simulink model "Test2D_Disks_in_Box"  (R2024a)
settings: Solver=ode15s  StartTime=0.0  StopTime=3  MaxStep=1e-2  RelTol=1e-4  AbsTol=1e-5  EnableMultiTasking=on
PostLoadFcn:
  | warning off Simulink:Engine:UsingDefaultMaxStepSize
InitFcn:
  | k_contact = 1e4;
  | b_contact = 1e1;
StartFcn:
  | tic;
StopFcn:
  | Elapsed_Sim_Time = toc;
  | disp(['Elapsed Sim Time = ' num2str(Elapsed_Sim_Time)]);
model workspace (MATLAB code in the model file):
  | Disk.radius = 0.05;
  | Disk.length = 0.01;
  | Disk.density = 1000;
  | 
  | Box.outer_width = 0.51*2;
  | Box.inner_width = 0.49*2;
  | Box.width = 0.05;
undefined symbols (not defined in the file or in its folder): Extr_Data_Box, X, Y, Z
libraries: sm_lib x22, Contact_Forces_Lib x15, Parts_Lib x3, nesl_utility x2
CloseFcn:
  | try,close(h1_Test2D_Disks_in_Box),end
  | clear h1_Test2D_Disks_in_Box
  | 
  | clear simlog_Test2D_Disks_in_Box
  | clear logsout_Test2D_Disks_in_Box
Description:
  | Test Model Disks in Box
  | 
  | Copyright 2015-2024 The MathWorks, Inc.
settings Model: Creator=smiller  LastModifiedBy=smiller
settings SolverCC: AutoScaleAbsTol=off  AlgebraicLoopSolver=TrustRegion
settings DataIOCC: MaxDataPoints=10000  SaveFormat=Array  ReturnWorkspaceOutputs=off  SignalLoggingName=logsout_Test2D_Disks_in_Box
settings OptimizationCC: ReuseModelBlockBuffer=off  ExpressionDepthLimit=2147483647  LifeSpan=inf
settings DebuggingCC: AlgebraicLoopMsg=error  UnderspecifiedInitializationDetection=Classic  MergeDetectMultiDrivingBlocksExec=none  IgnoredZcDiagnostic=none  SolverPrmCheckMsg=warning  FcnCallInpInsideContextMsg=warning  UnconnectedInputMsg=warning  UnconnectedLineMsg=warning  AllowSymbolicDim=off  StateNameClashWarn=warning  PregeneratedLibrarySubsystemCodeDiagnostic=none  SFUnexpectedBacktrackingDiag=warning  SFNoUnconditionalDefaultTransitionDiag=warning  SFExecutionAtInitializationDiag=none  ArithmeticOperatorsInVariantConditions=warning
settings HardwareCC: ProdBitPerPointer=32  ProdBitPerSizeT=32  ProdBitPerPtrDiffT=32  ProdLargestAtomicFloat=None  ProdIntDivRoundTo=Undefined  ProdEndianess=Unspecified  ProdWordSize=32  ProdHWDeviceType=32-bit Generic
settings ModelReferenceCC: EnableRefExpFcnMdlSchedulingChecks=on  PropagateSignalLabelsOutOfModel=off
settings SFSimCC: SimUseLocalCustomCode=off  CustomCodeUndefinedFunction=UseInterfaceOnly
settings RTWCC: RTWUseLocalCustomCode=off  GPUComputeCapability=3.5  DLArmComputeVersion=19.05
settings CodeAppCC: StateflowObjectComments=on
settings GRTTargetCC: TargetLangStandard=C89/C90 (ANSI)
settings ConfigComp: CovMetricSettings=dw  CovSaveCumulativeToWorkspaceVar=on  CovSaveSingleToWorkspaceVar=on  CovExternalEMLEnable=off  CovSFcnEnable=off
settings SimscapeCC: SimscapeNormalizeSystem=off  SimscapeLogType=all  SimscapeLogSimulationStatistics=on  SimscapeLogName=simlog_Test2D_Disks_in_Box  SimscapeLogDataHistory=10000
settings ConfigurationSet: Description=SimMechanics 2G
settings DiagnosticsConfigSet: SimMechanicsRigidlyBoundBlock=none
settings ExplorerConfigSet: InternalSimMechanicsExplorerSettings="<ExplorerConfiguration><canonicalview>default</canonicalview><AnimationSetting><BasePlaybackSpeed>1.0</BasePlaybackSpeed><PlaybackSpeedFactor>1.0</PlaybackSpeedFactor></AnimationSetting><TilePanel><TileInfo><Tiles Columns=\"1\" Count=\"1\" Rows=\"1\"><Column Left=\"2\" Weight=\"1\"/><Column Left=\"635\"/><Row Top=\"2\" Weight=\"1\"/><Row Top=\"394\"/><Tile Height=\"1\" Width=\"1\" X=\"0\" Y=\"0\"/></Tiles></TileInfo><SceneInfo><SceneViewer><BGColor><R>0.90588235855102539</R><G>0.94117647409439087</G><B>0.94117647409439087</B></BGColor><Camera><DoPerspective>off</DoPerspective><Position><X>0</X><Y>-1.0218563054680825</Y><Z>2.2204460492503131e-16</Z></Position><Center><X>0</X><Y>-4.9303806576313238e-32</Y><Z>2.2204460492503131e-16</Z></Center><Up><X>0</X><Y>-0</Y><Z>1</Z></Up><ViewLimDist>1</ViewLimDist><YLim>0.52529999017715456</YLim><XLim>0.85584123725990713</XLim></Camera></SceneViewer></SceneInfo></TilePanel><MechEditorPanel><Cameras/><GfxPanelCameraMap/></MechEditorPanel></ExplorerConfiguration>"

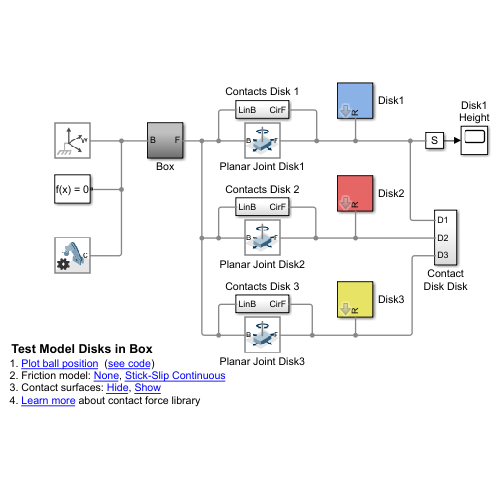
[thumbnail: Simulink's stored preview of the top-level diagram]
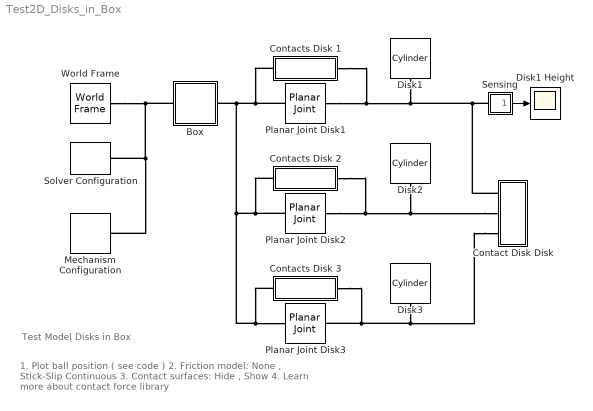
== system Test2D_Disks_in_Box ==
  note: 1. Plot ball position ( see code )
      | 2. Friction model: None , Stick-Slip Continuous
      | 3. Contact surfaces: Hide , Show
      | 4. Learn more about contact force library
  note: Test Model Disks in Box
  Box : Subsystem  Tag=CustomStyle
  Contact Disk Disk : Subsystem
  Contacts Disk 1 : Subsystem
  Contacts Disk 2 : Subsystem
  Contacts Disk 3 : Subsystem
  Disk1 : Parts_Lib/Cylinder  cyl_radius=Disk.radius  cyl_length=Disk.length  cyl_density=Disk.density  cyl_color=blue  cyl_opacity=1  cyl_color_custom="[0.7920    0.9900    0.9900]"  mark_radius=[0.75 0.5]  mark_len_factor=1.01  mark_angle=60  mark_color=orange  mark_opacity=1
  Disk1 Height : Scope
  Disk2 : Parts_Lib/Cylinder  cyl_radius=Disk.radius  cyl_length=Disk.length  cyl_density=Disk.density  cyl_color=red  cyl_opacity=1  cyl_color_custom="[0.7920    0.9900    0.9900]"  mark_radius=[0.75 0.5]  mark_len_factor=1.01  mark_angle=60  mark_color=green  mark_opacity=1
  Disk3 : Parts_Lib/Cylinder  cyl_radius=Disk.radius  cyl_length=Disk.length  cyl_density=Disk.density  cyl_color=yellow  cyl_opacity=1  cyl_color_custom="[0.7920    0.9900    0.9900]"  mark_radius=[0.75 0.5]  mark_len_factor=1.01  mark_angle=60  mark_color=purple  mark_opacity=1
  Mechanism Configuration : sm_lib/Utilities/Mechanism Configuration  UniformGravity=Constant  GravityVector=[0 0 -9.81]  GravityVectorUnits=m/s^2  LinearizationDelta=0.001  JointModeTransitionNonlinearIterations=2
  Planar Joint Disk1 : sm_lib/Joints/Planar Joint  JointMode=Normal  CompositeWrenchDir=FollowerOnBase  CompositeWrenchFrame=BaseFrame  SenseConstraintForce=off  SenseConstraintTorque=off  SenseTotalForce=off  SenseTotalTorque=off  PxPositionTargetSpecify=on  PxPositionTargetPriority=High  PxPositionTargetValue=0.3  PxPositionTargetValueUnits=m  PxVelocityTargetSpecify=on  PxVelocityTargetPriority=High  PxVelocityTargetValue=-1  PxVelocityTargetValueUnits=m/s  PxEquilibriumPosition=0  PxEquilibriumPositionUnits=m  PxSpringStiffness=0  PxSpringStiffnessUnits=N/m  PxDampingCoefficient=0  PxDampingCoefficientUnits=N/(m/s)  PxLowerLimitSpecify=off  PxLowerLimitBound=-1  PxLowerLimitBoundUnits=m  PxLowerLimitStiffness=1e6  PxLowerLimitStiffnessUnits=N/m  PxLowerLimitDamping=1e3  PxLowerLimitDampingUnits=N/(m/s)  PxLowerLimitTransitionRegionWidth=1e-4  PxLowerLimitTransitionRegionWidthUnits=m  PxUpperLimitSpecify=off  PxUpperLimitBound=1  PxUpperLimitBoundUnits=m  PxUpperLimitStiffness=1e6  PxUpperLimitStiffnessUnits=N/m  PxUpperLimitDamping=1e3  PxUpperLimitDampingUnits=N/(m/s)  PxUpperLimitTransitionRegionWidth=1e-4  PxUpperLimitTransitionRegionWidthUnits=m  PxTorqueActuationMode=NoTorque  PxMotionActuationMode=ComputedMotion  PxSensePosition=off  PxSenseVelocity=off  PxSenseAcceleration=off  PxSenseTorqueForce=off  PxSenseLowerLimitTorqueForce=off  PxSenseUpperLimitTorqueForce=off  PyPositionTargetSpecify=off  PyPositionTargetPriority=High  PyPositionTargetValue=0  PyPositionTargetValueUnits=m  PyVelocityTargetSpecify=on  PyVelocityTargetPriority=High  PyVelocityTargetValue=1  PyVelocityTargetValueUnits=m/s  PyEquilibriumPosition=0  PyEquilibriumPositionUnits=m  PySpringStiffness=0  PySpringStiffnessUnits=N/m  PyDampingCoefficient=0  PyDampingCoefficientUnits=N/(m/s)  PyLowerLimitSpecify=off  PyLowerLimitBound=-1  PyLowerLimitBoundUnits=m  PyLowerLimitStiffness=1e6  PyLowerLimitStiffnessUnits=N/m  PyLowerLimitDamping=1e3  PyLowerLimitDampingUnits=N/(m/s)  PyLowerLimitTransitionRegionWidth=1e-4  PyLowerLimitTransitionRegionWidthUnits=m  PyUpperLimitSpecify=off  PyUpperLimitBound=1  PyUpperLimitBoundUnits=m  PyUpperLimitStiffness=1e6  PyUpperLimitStiffnessUnits=N/m  PyUpperLimitDamping=1e3  PyUpperLimitDampingUnits=N/(m/s)  PyUpperLimitTransitionRegionWidth=1e-4  PyUpperLimitTransitionRegionWidthUnits=m  PyTorqueActuationMode=NoTorque  PyMotionActuationMode=ComputedMotion  PySensePosition=off  PySenseVelocity=off  PySenseAcceleration=off  PySenseTorqueForce=off  PySenseLowerLimitTorqueForce=off  PySenseUpperLimitTorqueForce=off  RzPositionTargetSpecify=off  RzPositionTargetPriority=High  RzPositionTargetValue=0  RzPositionTargetValueUnits=deg  RzVelocityTargetSpecify=off  RzVelocityTargetPriority=High  RzVelocityTargetValue=0  RzVelocityTargetValueUnits=deg/s  RzEquilibriumPosition=0  RzEquilibriumPositionUnits=deg  RzSpringStiffness=0  RzSpringStiffnessUnits=N*m/deg  RzDampingCoefficient=0  RzDampingCoefficientUnits=N*m/(deg/s)  RzLowerLimitSpecify=off  RzLowerLimitBound=-90  RzLowerLimitBoundUnits=deg  RzLowerLimitStiffness=1e4  RzLowerLimitStiffnessUnits=N*m/deg  RzLowerLimitDamping=10  RzLowerLimitDampingUnits=N*m/(deg/s)  RzLowerLimitTransitionRegionWidth=0.1  RzLowerLimitTransitionRegionWidthUnits=deg  RzUpperLimitSpecify=off  RzUpperLimitBound=90  RzUpperLimitBoundUnits=deg  RzUpperLimitStiffness=1e4  RzUpperLimitStiffnessUnits=N*m/deg  RzUpperLimitDamping=10  RzUpperLimitDampingUnits=N*m/(deg/s)  RzUpperLimitTransitionRegionWidth=0.1  RzUpperLimitTransitionRegionWidthUnits=deg  RzTorqueActuationMode=NoTorque  RzMotionActuationMode=ComputedMotion  RzSensePosition=off  RzSenseVelocity=off  RzSenseAcceleration=off  RzSenseTorqueForce=off  RzSenseLowerLimitTorqueForce=off  RzSenseUpperLimitTorqueForce=off
  Planar Joint Disk2 : sm_lib/Joints/Planar Joint  JointMode=Normal  CompositeWrenchDir=FollowerOnBase  CompositeWrenchFrame=BaseFrame  SenseConstraintForce=off  SenseConstraintTorque=off  SenseTotalForce=off  SenseTotalTorque=off  PxPositionTargetSpecify=on  PxPositionTargetPriority=High  PxPositionTargetValue=-0.3  PxPositionTargetValueUnits=m  PxVelocityTargetSpecify=on  PxVelocityTargetPriority=High  PxVelocityTargetValue=+1  PxVelocityTargetValueUnits=m/s  PxEquilibriumPosition=0  PxEquilibriumPositionUnits=m  PxSpringStiffness=0  PxSpringStiffnessUnits=N/m  PxDampingCoefficient=0  PxDampingCoefficientUnits=N/(m/s)  PxLowerLimitSpecify=off  PxLowerLimitBound=-1  PxLowerLimitBoundUnits=m  PxLowerLimitStiffness=1e6  PxLowerLimitStiffnessUnits=N/m  PxLowerLimitDamping=1e3  PxLowerLimitDampingUnits=N/(m/s)  PxLowerLimitTransitionRegionWidth=1e-4  PxLowerLimitTransitionRegionWidthUnits=m  PxUpperLimitSpecify=off  PxUpperLimitBound=1  PxUpperLimitBoundUnits=m  PxUpperLimitStiffness=1e6  PxUpperLimitStiffnessUnits=N/m  PxUpperLimitDamping=1e3  PxUpperLimitDampingUnits=N/(m/s)  PxUpperLimitTransitionRegionWidth=1e-4  PxUpperLimitTransitionRegionWidthUnits=m  PxTorqueActuationMode=NoTorque  PxMotionActuationMode=ComputedMotion  PxSensePosition=off  PxSenseVelocity=off  PxSenseAcceleration=off  PxSenseTorqueForce=off  PxSenseLowerLimitTorqueForce=off  PxSenseUpperLimitTorqueForce=off  PyPositionTargetSpecify=off  PyPositionTargetPriority=High  PyPositionTargetValue=0  PyPositionTargetValueUnits=m  PyVelocityTargetSpecify=on  PyVelocityTargetPriority=High  PyVelocityTargetValue=-0.8  PyVelocityTargetValueUnits=m/s  PyEquilibriumPosition=0  PyEquilibriumPositionUnits=m  PySpringStiffness=0  PySpringStiffnessUnits=N/m  PyDampingCoefficient=0  PyDampingCoefficientUnits=N/(m/s)  PyLowerLimitSpecify=off  PyLowerLimitBound=-1  PyLowerLimitBoundUnits=m  PyLowerLimitStiffness=1e6  PyLowerLimitStiffnessUnits=N/m  PyLowerLimitDamping=1e3  PyLowerLimitDampingUnits=N/(m/s)  PyLowerLimitTransitionRegionWidth=1e-4  PyLowerLimitTransitionRegionWidthUnits=m  PyUpperLimitSpecify=off  PyUpperLimitBound=1  PyUpperLimitBoundUnits=m  PyUpperLimitStiffness=1e6  PyUpperLimitStiffnessUnits=N/m  PyUpperLimitDamping=1e3  PyUpperLimitDampingUnits=N/(m/s)  PyUpperLimitTransitionRegionWidth=1e-4  PyUpperLimitTransitionRegionWidthUnits=m  PyTorqueActuationMode=NoTorque  PyMotionActuationMode=ComputedMotion  PySensePosition=off  PySenseVelocity=off  PySenseAcceleration=off  PySenseTorqueForce=off  PySenseLowerLimitTorqueForce=off  PySenseUpperLimitTorqueForce=off  RzPositionTargetSpecify=off  RzPositionTargetPriority=High  RzPositionTargetValue=0  RzPositionTargetValueUnits=deg  RzVelocityTargetSpecify=off  RzVelocityTargetPriority=High  RzVelocityTargetValue=0  RzVelocityTargetValueUnits=deg/s  RzEquilibriumPosition=0  RzEquilibriumPositionUnits=deg  RzSpringStiffness=0  RzSpringStiffnessUnits=N*m/deg  RzDampingCoefficient=0  RzDampingCoefficientUnits=N*m/(deg/s)  RzLowerLimitSpecify=off  RzLowerLimitBound=-90  RzLowerLimitBoundUnits=deg  RzLowerLimitStiffness=1e4  RzLowerLimitStiffnessUnits=N*m/deg  RzLowerLimitDamping=10  RzLowerLimitDampingUnits=N*m/(deg/s)  RzLowerLimitTransitionRegionWidth=0.1  RzLowerLimitTransitionRegionWidthUnits=deg  RzUpperLimitSpecify=off  RzUpperLimitBound=90  RzUpperLimitBoundUnits=deg  RzUpperLimitStiffness=1e4  RzUpperLimitStiffnessUnits=N*m/deg  RzUpperLimitDamping=10  RzUpperLimitDampingUnits=N*m/(deg/s)  RzUpperLimitTransitionRegionWidth=0.1  RzUpperLimitTransitionRegionWidthUnits=deg  RzTorqueActuationMode=NoTorque  RzMotionActuationMode=ComputedMotion  RzSensePosition=off  RzSenseVelocity=off  RzSenseAcceleration=off  RzSenseTorqueForce=off  RzSenseLowerLimitTorqueForce=off  RzSenseUpperLimitTorqueForce=off
  Planar Joint Disk3 : sm_lib/Joints/Planar Joint  JointMode=Normal  CompositeWrenchDir=FollowerOnBase  CompositeWrenchFrame=BaseFrame  SenseConstraintForce=off  SenseConstraintTorque=off  SenseTotalForce=off  SenseTotalTorque=off  PxPositionTargetSpecify=off  PxPositionTargetPriority=High  PxPositionTargetValue=0  PxPositionTargetValueUnits=m  PxVelocityTargetSpecify=on  PxVelocityTargetPriority=High  PxVelocityTargetValue=+1  PxVelocityTargetValueUnits=m/s  PxEquilibriumPosition=0  PxEquilibriumPositionUnits=m  PxSpringStiffness=0  PxSpringStiffnessUnits=N/m  PxDampingCoefficient=0  PxDampingCoefficientUnits=N/(m/s)  PxLowerLimitSpecify=off  PxLowerLimitBound=-1  PxLowerLimitBoundUnits=m  PxLowerLimitStiffness=1e6  PxLowerLimitStiffnessUnits=N/m  PxLowerLimitDamping=1e3  PxLowerLimitDampingUnits=N/(m/s)  PxLowerLimitTransitionRegionWidth=1e-4  PxLowerLimitTransitionRegionWidthUnits=m  PxUpperLimitSpecify=off  PxUpperLimitBound=1  PxUpperLimitBoundUnits=m  PxUpperLimitStiffness=1e6  PxUpperLimitStiffnessUnits=N/m  PxUpperLimitDamping=1e3  PxUpperLimitDampingUnits=N/(m/s)  PxUpperLimitTransitionRegionWidth=1e-4  PxUpperLimitTransitionRegionWidthUnits=m  PxTorqueActuationMode=NoTorque  PxMotionActuationMode=ComputedMotion  PxSensePosition=off  PxSenseVelocity=off  PxSenseAcceleration=off  PxSenseTorqueForce=off  PxSenseLowerLimitTorqueForce=off  PxSenseUpperLimitTorqueForce=off  PyPositionTargetSpecify=on  PyPositionTargetPriority=High  PyPositionTargetValue=0.3  PyPositionTargetValueUnits=m  PyVelocityTargetSpecify=on  PyVelocityTargetPriority=High  PyVelocityTargetValue=-0.8  PyVelocityTargetValueUnits=m/s  PyEquilibriumPosition=0  PyEquilibriumPositionUnits=m  PySpringStiffness=0  PySpringStiffnessUnits=N/m  PyDampingCoefficient=0  PyDampingCoefficientUnits=N/(m/s)  PyLowerLimitSpecify=off  PyLowerLimitBound=-1  PyLowerLimitBoundUnits=m  PyLowerLimitStiffness=1e6  PyLowerLimitStiffnessUnits=N/m  PyLowerLimitDamping=1e3  PyLowerLimitDampingUnits=N/(m/s)  PyLowerLimitTransitionRegionWidth=1e-4  PyLowerLimitTransitionRegionWidthUnits=m  PyUpperLimitSpecify=off  PyUpperLimitBound=1  PyUpperLimitBoundUnits=m  PyUpperLimitStiffness=1e6  PyUpperLimitStiffnessUnits=N/m  PyUpperLimitDamping=1e3  PyUpperLimitDampingUnits=N/(m/s)  PyUpperLimitTransitionRegionWidth=1e-4  PyUpperLimitTransitionRegionWidthUnits=m  PyTorqueActuationMode=NoTorque  PyMotionActuationMode=ComputedMotion  PySensePosition=off  PySenseVelocity=off  PySenseAcceleration=off  PySenseTorqueForce=off  PySenseLowerLimitTorqueForce=off  PySenseUpperLimitTorqueForce=off  RzPositionTargetSpecify=off  RzPositionTargetPriority=High  RzPositionTargetValue=0  RzPositionTargetValueUnits=deg  RzVelocityTargetSpecify=off  RzVelocityTargetPriority=High  RzVelocityTargetValue=0  RzVelocityTargetValueUnits=deg/s  RzEquilibriumPosition=0  RzEquilibriumPositionUnits=deg  RzSpringStiffness=0  RzSpringStiffnessUnits=N*m/deg  RzDampingCoefficient=0  RzDampingCoefficientUnits=N*m/(deg/s)  RzLowerLimitSpecify=off  RzLowerLimitBound=-90  RzLowerLimitBoundUnits=deg  RzLowerLimitStiffness=1e4  RzLowerLimitStiffnessUnits=N*m/deg  RzLowerLimitDamping=10  RzLowerLimitDampingUnits=N*m/(deg/s)  RzLowerLimitTransitionRegionWidth=0.1  RzLowerLimitTransitionRegionWidthUnits=deg  RzUpperLimitSpecify=off  RzUpperLimitBound=90  RzUpperLimitBoundUnits=deg  RzUpperLimitStiffness=1e4  RzUpperLimitStiffnessUnits=N*m/deg  RzUpperLimitDamping=10  RzUpperLimitDampingUnits=N*m/(deg/s)  RzUpperLimitTransitionRegionWidth=0.1  RzUpperLimitTransitionRegionWidthUnits=deg  RzTorqueActuationMode=NoTorque  RzMotionActuationMode=ComputedMotion  RzSensePosition=off  RzSenseVelocity=off  RzSenseAcceleration=off  RzSenseTorqueForce=off  RzSenseLowerLimitTorqueForce=off  RzSenseUpperLimitTorqueForce=off
  Sensing : Subsystem
      mask Display: disp('S')
  Solver Configuration : nesl_utility/Solver Configuration  PhysicalDomain=network_engine_domain  SubClassName=solver  LeftPortType=input  RightPortType=generic  Tones=[]  Harmonics=[]  SimulateNoise=off  Profile=off  UseLocalSampling=off  EnableSwitchedLinearOptims=on  FrequencyDomain=off  UseCCode=off  RelTol=0.001  AbsTol=1e-06  MinStep=1e-09  ToWorkspace=off  RevertToSquareIcSolve=off  NumHomotopyIterations=100  PhasorMode=off  PhasorModeNumHarmonics=1  ConsistencySolver=NEWTON_FTOL  IndexReductionMethod=DerivativeReplacement  DoDC=off  ResidualTolerance=1e-9  ConsistencyTolSource=GLOBAL  ConsistencyAbsTol=0.001  ConsistencyRelTol=0.001  ConsistencyTolFactor=0.001  UseLocalSolver=off  LocalSolverChoice=NE_BACKWARD_EULER_ADVANCER  ResolveIndetEquations=on  FunctionEvalNumThread=1  LocalSolverSampleTime=.001  DoFixedCost=off  MaxNonlinIter=3  MaxModeIter=2  ComputeImpulses=off  ImpulseIterations=2  LinearAlgebra=Sparse  LinearAlgebraNumThread=0  EquationFormulation=NE_TIME_EF  DelaysMemoryBudget=1024  AutomaticFiltering=on  FilteringTimeConstant=0.001  PartitionStorageMethod=AS_NEEDED  PartitionMemoryBudget=1024  PartitionMethod=FAST  MultibodyUseLocalSolver=off  MultibodyLocalSolverChoice=ODE1  MultibodyLocalSolverSampleTime=0.001
  World Frame : sm_lib/Frames and Transforms/World Frame
  wires:
  Sensing/1(S) -> Disk1 Height/1
  connections:
  Contact Disk Disk/LConn2 -- Disk2/LConn1 -- Contacts Disk 2/LConn1 -- Planar Joint Disk2/RConn1
  Contact Disk Disk/LConn1 -- Disk1/LConn1 -- Contacts Disk 1/LConn1 -- Planar Joint Disk1/RConn1 -- Sensing/LConn1
  Mechanism Configuration/RConn1 -- Solver Configuration/RConn1 -- Box/LConn1 -- World Frame/RConn1
  Contact Disk Disk/LConn3 -- Disk3/LConn1 -- Contacts Disk 3/LConn1 -- Planar Joint Disk3/RConn1
  Planar Joint Disk1/LConn1 -- Contacts Disk 1/RConn1 -- Contacts Disk 3/RConn1 -- Planar Joint Disk3/LConn1 -- Contacts Disk 2/RConn1 -- Planar Joint Disk2/LConn1 -- Box/RConn1

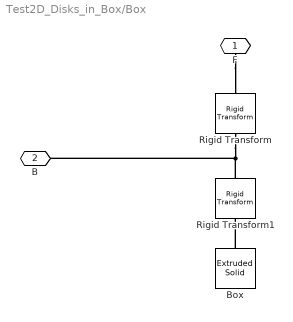
== system Test2D_Disks_in_Box/Box ==
  Box : sm_lib/Body Elements/Extruded Solid  ExtrusionType=General  PolygonNumSides=3  PolygonOuterRadius=1  PolygonOuterRadiusUnits=m  ExportEntireGeometry=off  ExtrusionCrossSection=Extr_Data_Box(Box.outer_width,Box.inner_width)  ExtrusionCrossSectionUnits=m  ExportConvexHullGeometry=off  ExtrusionLength=Box.width  ExtrusionLengthUnits=m  InertiaType=CalculateFromGeometry  BasedOnType=Density  Density=1000  DensityUnits=kg/(m^3)  Mass=1  MassUnits=kg  CenterOfMass=[0 0 0]  CenterOfMassUnits=m  MomentsOfInertia=[1 1 1]  MomentsOfInertiaUnits=kg*m^2  ProductsOfInertia=[0 0 0]  ProductsOfInertiaUnits=kg*m^2  GraphicType=FromGeometry  MarkerShape=Sphere  MarkerSize=10  GraphicVisPropType=SimpleVisualProperties  GraphicDiffuseColor=[0.5 0.5 0.5]  GraphicOpacity=1.0  GraphicSpecularColor=[0.5 0.5 0.5 1.0]  GraphicAmbientColor=[0.15 0.15 0.15 1.0]  GraphicEmissiveColor=[0.0 0.0 0.0 1.0]  GraphicShininess=75  DoExposeReferenceFrame=on  SerializedFrames=<Frames/>
  Rigid Transform : sm_lib/Frames and Transforms/Rigid Transform  RotationMethod=AlignedAxes  FollAlignAxisA=+X  BaseAlignAxisA=+Z  FollAlignAxisB=+Y  BaseAlignAxisB=+X  RotationStandardAxis=+Z  RotationAngle=0  RotationAngleUnits=deg  RotationArbitraryAxis=[0 0 1]  RotationSequenceAxes=FollowerAxes  RotationSequence=XYX  RotationSequenceAngles=[0 0 0]  RotationSequenceAnglesUnits=deg  RotationMatrix=[1 0 0; 0 1 0; 0 0 1]  Quaternion=[1 0 0 0]  TranslationMethod=None  TranslationCartesianOffset=[0 0 0]  TranslationCartesianOffsetUnits=m  TranslationStandardAxis=+Z  TranslationStandardOffset=0  TranslationStandardOffsetUnits=m  TranslationROffset=0  TranslationROffsetUnits=m  TranslationThetaOffset=0  TranslationThetaOffsetUnits=deg  TranslationZOffset=0  TranslationZOffsetUnits=m
  Rigid Transform1 : sm_lib/Frames and Transforms/Rigid Transform  RotationMethod=StandardAxis  FollAlignAxisA=+X  BaseAlignAxisA=+Z  FollAlignAxisB=+Y  BaseAlignAxisB=+X  RotationStandardAxis=+X  RotationAngle=90  RotationAngleUnits=deg  RotationArbitraryAxis=[0 0 1]  RotationSequenceAxes=FollowerAxes  RotationSequence=XYX  RotationSequenceAngles=[0 0 0]  RotationSequenceAnglesUnits=deg  RotationMatrix=[1 0 0; 0 1 0; 0 0 1]  Quaternion=[1 0 0 0]  TranslationMethod=None  TranslationCartesianOffset=[0 0 0]  TranslationCartesianOffsetUnits=m  TranslationStandardAxis=+Z  TranslationStandardOffset=0  TranslationStandardOffsetUnits=m  TranslationROffset=0  TranslationROffsetUnits=m  TranslationThetaOffset=0  TranslationThetaOffsetUnits=deg  TranslationZOffset=0  TranslationZOffsetUnits=m
  F : PMIOPort  Side=Right
  B : PMIOPort  Port=2  Side=Left
  connections:
  F/RConn1 -- Rigid Transform/RConn1
  Box/RConn1 -- Rigid Transform1/RConn1
  Rigid Transform/LConn1 -- B/RConn1 -- Rigid Transform1/LConn1

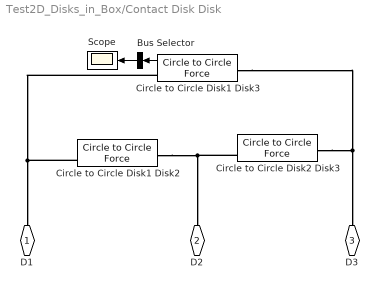
== system Test2D_Disks_in_Box/Contact Disk Disk ==
  Bus Selector : BusSelector  OutputSignals=Spr Force,Damp Force  OutputAsBus=on
  Circle to Circle Disk1 Disk2 : Contact_Forces_Lib/2D/Circle to Circle Force  cirB_rad=Disk.radius  cirF_rad=Disk.radius  active_angle=[-180 180]  force_law=Linear  k_contact=k_contact  b_contact=b_contact  pen_full_damp_F=1e-4  pen_exponent=1  custom_param_1=1  custom_param_2=1  friction_law=None  mu_kinetic=0.5  mu_static=0.7  v_thr=0.001  vis_on=off  vis_opc_en=0  vis_len_cirBz=Disk.length*1.05  vis_len_cirBx=Disk.radius*0.05  vis_len_cirFz=Disk.length*1.05  vis_len_cirFx=Disk.radius*0.05  vis_clr=[0.9 0.2 0.2]  vis_opc=0.7
  Circle to Circle Disk1 Disk3 : Contact_Forces_Lib/2D/Circle to Circle Force  cirB_rad=Disk.radius  cirF_rad=Disk.radius  active_angle=[-180 180]  force_law=Linear  k_contact=k_contact  b_contact=b_contact  pen_full_damp_F=1e-4  pen_exponent=1  custom_param_1=1  custom_param_2=1  friction_law=None  mu_kinetic=0.5  mu_static=0.7  v_thr=0.001  vis_on=off  vis_opc_en=0  vis_len_cirBz=Disk.length*1.05  vis_len_cirBx=Disk.radius*0.05  vis_len_cirFz=Disk.length*1.05  vis_len_cirFx=Disk.radius*0.05  vis_clr=[0.9 0.2 0.2]  vis_opc=0.7
  Circle to Circle Disk2 Disk3 : Contact_Forces_Lib/2D/Circle to Circle Force  cirB_rad=Disk.radius  cirF_rad=Disk.radius  active_angle=[-180 180]  force_law=Linear  k_contact=k_contact  b_contact=b_contact  pen_full_damp_F=1e-4  pen_exponent=1  custom_param_1=1  custom_param_2=1  friction_law=None  mu_kinetic=0.5  mu_static=0.7  v_thr=0.001  vis_on=off  vis_opc_en=0  vis_len_cirBz=Disk.length*1.05  vis_len_cirBx=Disk.radius*0.05  vis_len_cirFz=Disk.length*1.05  vis_len_cirFx=Disk.radius*0.05  vis_clr=[0.9 0.2 0.2]  vis_opc=0.7
  Scope : Scope
  D1 : PMIOPort  Side=Left
  D2 : PMIOPort  Port=2  Side=Left
  D3 : PMIOPort  Port=3  Side=Left
  wires:
  Circle to Circle Disk1 Disk3/1 -> Bus Selector/1
  Bus Selector/1 -> Scope/1
  connections:
  Circle to Circle Disk1 Disk3/RConn1 -- Circle to Circle Disk1 Disk2/RConn1 -- D1/RConn1
  Circle to Circle Disk2 Disk3/RConn1 -- Circle to Circle Disk1 Disk2/LConn1 -- D2/RConn1
  Circle to Circle Disk2 Disk3/LConn1 -- Circle to Circle Disk1 Disk3/LConn1 -- D3/RConn1

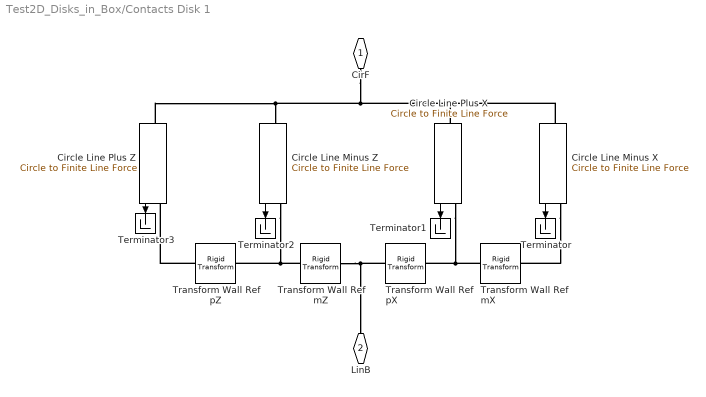
== system Test2D_Disks_in_Box/Contacts Disk 1 ==
  Circle Line Minus X : Contact_Forces_Lib/2D/Circle to Finite Line Force  circle_rad=Disk.radius  line_depth=(Box.outer_width/2-Box.inner_width/2)/2  line_length=(Box.outer_width+Box.inner_width)/2  force_law=Linear  k_contact=k_contact  b_contact=b_contact  pen_full_damp_F=1e-4  pen_exponent=1  custom_param_1=1  custom_param_2=1  friction_law=None  mu_kinetic=0.5  mu_static=0.7  v_thr=0.001  vis_on=off  vis_opc_en=0  vis_len_linBz=Box.width*1.05  vis_len_linBx=Box.outer_width*0.005  vis_len_cirFz=Disk.length*1.05  vis_len_cirFx=Disk.radius*0.05  vis_clr=[0.9 0.2 0.2]  vis_opc=0.7
  Circle Line Minus Z : Contact_Forces_Lib/2D/Circle to Finite Line Force  circle_rad=Disk.radius  line_depth=(Box.outer_width/2-Box.inner_width/2)/2  line_length=(Box.outer_width+Box.inner_width)/2  force_law=Linear  k_contact=k_contact  b_contact=b_contact  pen_full_damp_F=1e-4  pen_exponent=1  custom_param_1=1  custom_param_2=1  friction_law=None  mu_kinetic=0.5  mu_static=0.7  v_thr=0.001  vis_on=off  vis_opc_en=0  vis_len_linBz=Box.width*1.05  vis_len_linBx=Box.outer_width*0.005  vis_len_cirFz=Disk.length*1.05  vis_len_cirFx=Disk.radius*0.05  vis_clr=[0.9 0.2 0.2]  vis_opc=0.7
  Circle Line Plus X : Contact_Forces_Lib/2D/Circle to Finite Line Force  circle_rad=Disk.radius  line_depth=(Box.outer_width/2-Box.inner_width/2)/2  line_length=(Box.outer_width+Box.inner_width)/2  force_law=Linear  k_contact=k_contact  b_contact=b_contact  pen_full_damp_F=1e-4  pen_exponent=1  custom_param_1=1  custom_param_2=1  friction_law=None  mu_kinetic=0.5  mu_static=0.7  v_thr=0.001  vis_on=off  vis_opc_en=0  vis_len_linBz=Box.width*1.05  vis_len_linBx=Box.outer_width*0.005  vis_len_cirFz=Disk.length*1.05  vis_len_cirFx=Disk.radius*0.05  vis_clr=[0.9 0.2 0.2]  vis_opc=0.7
  Circle Line Plus Z : Contact_Forces_Lib/2D/Circle to Finite Line Force  circle_rad=Disk.radius  line_depth=(Box.outer_width/2-Box.inner_width/2)/2  line_length=(Box.outer_width+Box.inner_width)/2  force_law=Linear  k_contact=k_contact  b_contact=b_contact  pen_full_damp_F=1e-4  pen_exponent=1  custom_param_1=1  custom_param_2=1  friction_law=None  mu_kinetic=0.5  mu_static=0.7  v_thr=0.001  vis_on=off  vis_opc_en=0  vis_len_linBz=Box.width*1.05  vis_len_linBx=Box.outer_width*0.005  vis_len_cirFz=Disk.length*1.05  vis_len_cirFx=Disk.radius*0.05  vis_clr=[0.9 0.2 0.2]  vis_opc=0.7
  Terminator{,1..3} (4 alike) : Terminator
  Transform Wall Ref mX : sm_lib/Frames and Transforms/Rigid Transform  RotationMethod=StandardAxis  FollAlignAxisA=+X  BaseAlignAxisA=+Y  FollAlignAxisB=+Y  BaseAlignAxisB=+Z  RotationStandardAxis=+Z  RotationAngle=180  RotationAngleUnits=deg  RotationArbitraryAxis=[0 0 1]  RotationSequenceAxes=FollowerAxes  RotationSequence=XYX  RotationSequenceAngles=[0 0 0]  RotationSequenceAnglesUnits=deg  RotationMatrix=[1 0 0; 0 1 0; 0 0 1]  Quaternion=[1 0 0 0]  TranslationMethod=StandardAxis  TranslationCartesianOffset=[0 0 0]  TranslationCartesianOffsetUnits=m  TranslationStandardAxis=+X  TranslationStandardOffset=1  TranslationStandardOffsetUnits=m  TranslationROffset=0  TranslationROffsetUnits=m  TranslationThetaOffset=0  TranslationThetaOffsetUnits=deg  TranslationZOffset=0  TranslationZOffsetUnits=m
  Transform Wall Ref mZ : sm_lib/Frames and Transforms/Rigid Transform  RotationMethod=None  FollAlignAxisA=+X  BaseAlignAxisA=+Y  FollAlignAxisB=+Y  BaseAlignAxisB=+Z  RotationStandardAxis=+Z  RotationAngle=180  RotationAngleUnits=deg  RotationArbitraryAxis=[0 0 1]  RotationSequenceAxes=FollowerAxes  RotationSequence=XYX  RotationSequenceAngles=[0 0 0]  RotationSequenceAnglesUnits=deg  RotationMatrix=[1 0 0; 0 1 0; 0 0 1]  Quaternion=[1 0 0 0]  TranslationMethod=StandardAxis  TranslationCartesianOffset=[0 0 0]  TranslationCartesianOffsetUnits=m  TranslationStandardAxis=+X  TranslationStandardOffset=-0.5  TranslationStandardOffsetUnits=m  TranslationROffset=0  TranslationROffsetUnits=m  TranslationThetaOffset=0  TranslationThetaOffsetUnits=deg  TranslationZOffset=0  TranslationZOffsetUnits=m
  Transform Wall Ref pX : sm_lib/Frames and Transforms/Rigid Transform  RotationMethod=StandardAxis  FollAlignAxisA=+X  BaseAlignAxisA=+Y  FollAlignAxisB=+Y  BaseAlignAxisB=+Z  RotationStandardAxis=+Z  RotationAngle=-90  RotationAngleUnits=deg  RotationArbitraryAxis=[0 0 1]  RotationSequenceAxes=FollowerAxes  RotationSequence=XYX  RotationSequenceAngles=[0 0 0]  RotationSequenceAnglesUnits=deg  RotationMatrix=[1 0 0; 0 1 0; 0 0 1]  Quaternion=[1 0 0 0]  TranslationMethod=StandardAxis  TranslationCartesianOffset=[0 0 0]  TranslationCartesianOffsetUnits=m  TranslationStandardAxis=+Y  TranslationStandardOffset=0.5  TranslationStandardOffsetUnits=m  TranslationROffset=0  TranslationROffsetUnits=m  TranslationThetaOffset=0  TranslationThetaOffsetUnits=deg  TranslationZOffset=0  TranslationZOffsetUnits=m
  Transform Wall Ref pZ : sm_lib/Frames and Transforms/Rigid Transform  RotationMethod=StandardAxis  FollAlignAxisA=+X  BaseAlignAxisA=+Y  FollAlignAxisB=+Y  BaseAlignAxisB=+Z  RotationStandardAxis=+Z  RotationAngle=180  RotationAngleUnits=deg  RotationArbitraryAxis=[0 0 1]  RotationSequenceAxes=FollowerAxes  RotationSequence=XYX  RotationSequenceAngles=[0 0 0]  RotationSequenceAnglesUnits=deg  RotationMatrix=[1 0 0; 0 1 0; 0 0 1]  Quaternion=[1 0 0 0]  TranslationMethod=StandardAxis  TranslationCartesianOffset=[0 0 0]  TranslationCartesianOffsetUnits=m  TranslationStandardAxis=+X  TranslationStandardOffset=1  TranslationStandardOffsetUnits=m  TranslationROffset=0  TranslationROffsetUnits=m  TranslationThetaOffset=0  TranslationThetaOffsetUnits=deg  TranslationZOffset=0  TranslationZOffsetUnits=m
  CirF : PMIOPort  Side=Left
  LinB : PMIOPort  Port=2  Side=Right
  wires:
  Circle Line Minus Z/1 -> Terminator2/1
  Circle Line Minus X/1 -> Terminator/1
  Circle Line Plus X/1 -> Terminator1/1
  Circle Line Plus Z/1 -> Terminator3/1
  connections:
  CirF/RConn1 -- Circle Line Minus X/LConn1 -- Circle Line Plus X/LConn1 -- Circle Line Plus Z/LConn1 -- Circle Line Minus Z/LConn1
  Circle Line Minus Z/RConn1 -- Transform Wall Ref pZ/LConn1 -- Transform Wall Ref mZ/RConn1
  Transform Wall Ref pZ/RConn1 -- Circle Line Plus Z/RConn1
  Transform Wall Ref mZ/LConn1 -- Transform Wall Ref pX/LConn1 -- LinB/RConn1
  Circle Line Plus X/RConn1 -- Transform Wall Ref mX/LConn1 -- Transform Wall Ref pX/RConn1
  Circle Line Minus X/RConn1 -- Transform Wall Ref mX/RConn1

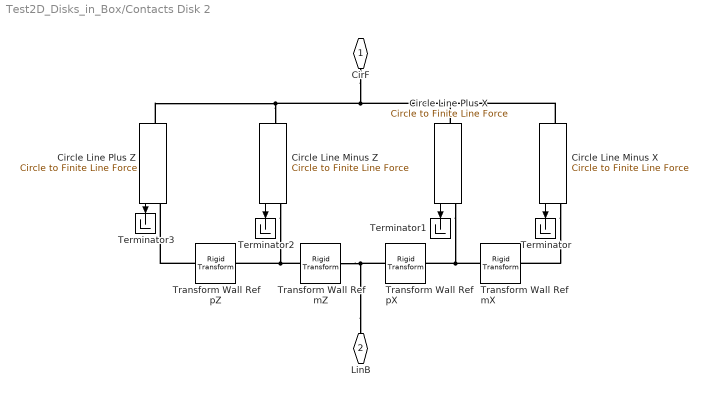
== system Test2D_Disks_in_Box/Contacts Disk 2 ==
  Circle Line Minus X : Contact_Forces_Lib/2D/Circle to Finite Line Force  circle_rad=Disk.radius  line_depth=(Box.outer_width/2-Box.inner_width/2)/2  line_length=(Box.outer_width+Box.inner_width)/2  force_law=Linear  k_contact=k_contact  b_contact=b_contact  pen_full_damp_F=1e-4  pen_exponent=1  custom_param_1=1  custom_param_2=1  friction_law=None  mu_kinetic=0.5  mu_static=0.7  v_thr=0.001  vis_on=off  vis_opc_en=0  vis_len_linBz=Box.width*1.05  vis_len_linBx=Box.outer_width*0.005  vis_len_cirFz=Disk.length*1.05  vis_len_cirFx=Disk.radius*0.05  vis_clr=[0.9 0.2 0.2]  vis_opc=0.7
  Circle Line Minus Z : Contact_Forces_Lib/2D/Circle to Finite Line Force  circle_rad=Disk.radius  line_depth=(Box.outer_width/2-Box.inner_width/2)/2  line_length=(Box.outer_width+Box.inner_width)/2  force_law=Linear  k_contact=k_contact  b_contact=b_contact  pen_full_damp_F=1e-4  pen_exponent=1  custom_param_1=1  custom_param_2=1  friction_law=None  mu_kinetic=0.5  mu_static=0.7  v_thr=0.001  vis_on=off  vis_opc_en=0  vis_len_linBz=Box.width*1.05  vis_len_linBx=Box.outer_width*0.005  vis_len_cirFz=Disk.length*1.05  vis_len_cirFx=Disk.radius*0.05  vis_clr=[0.9 0.2 0.2]  vis_opc=0.7
  Circle Line Plus X : Contact_Forces_Lib/2D/Circle to Finite Line Force  circle_rad=Disk.radius  line_depth=(Box.outer_width/2-Box.inner_width/2)/2  line_length=(Box.outer_width+Box.inner_width)/2  force_law=Linear  k_contact=k_contact  b_contact=b_contact  pen_full_damp_F=1e-4  pen_exponent=1  custom_param_1=1  custom_param_2=1  friction_law=None  mu_kinetic=0.5  mu_static=0.7  v_thr=0.001  vis_on=off  vis_opc_en=0  vis_len_linBz=Box.width*1.05  vis_len_linBx=Box.outer_width*0.005  vis_len_cirFz=Disk.length*1.05  vis_len_cirFx=Disk.radius*0.05  vis_clr=[0.9 0.2 0.2]  vis_opc=0.7
  Circle Line Plus Z : Contact_Forces_Lib/2D/Circle to Finite Line Force  circle_rad=Disk.radius  line_depth=(Box.outer_width/2-Box.inner_width/2)/2  line_length=(Box.outer_width+Box.inner_width)/2  force_law=Linear  k_contact=k_contact  b_contact=b_contact  pen_full_damp_F=1e-4  pen_exponent=1  custom_param_1=1  custom_param_2=1  friction_law=None  mu_kinetic=0.5  mu_static=0.7  v_thr=0.001  vis_on=off  vis_opc_en=0  vis_len_linBz=Box.width*1.05  vis_len_linBx=Box.outer_width*0.005  vis_len_cirFz=Disk.length*1.05  vis_len_cirFx=Disk.radius*0.05  vis_clr=[0.9 0.2 0.2]  vis_opc=0.7
  Terminator{,1..3} (4 alike) : Terminator
  Transform Wall Ref mX : sm_lib/Frames and Transforms/Rigid Transform  RotationMethod=StandardAxis  FollAlignAxisA=+X  BaseAlignAxisA=+Y  FollAlignAxisB=+Y  BaseAlignAxisB=+Z  RotationStandardAxis=+Z  RotationAngle=180  RotationAngleUnits=deg  RotationArbitraryAxis=[0 0 1]  RotationSequenceAxes=FollowerAxes  RotationSequence=XYX  RotationSequenceAngles=[0 0 0]  RotationSequenceAnglesUnits=deg  RotationMatrix=[1 0 0; 0 1 0; 0 0 1]  Quaternion=[1 0 0 0]  TranslationMethod=StandardAxis  TranslationCartesianOffset=[0 0 0]  TranslationCartesianOffsetUnits=m  TranslationStandardAxis=+X  TranslationStandardOffset=1  TranslationStandardOffsetUnits=m  TranslationROffset=0  TranslationROffsetUnits=m  TranslationThetaOffset=0  TranslationThetaOffsetUnits=deg  TranslationZOffset=0  TranslationZOffsetUnits=m
  Transform Wall Ref mZ : sm_lib/Frames and Transforms/Rigid Transform  RotationMethod=None  FollAlignAxisA=+X  BaseAlignAxisA=+Y  FollAlignAxisB=+Y  BaseAlignAxisB=+Z  RotationStandardAxis=+Z  RotationAngle=180  RotationAngleUnits=deg  RotationArbitraryAxis=[0 0 1]  RotationSequenceAxes=FollowerAxes  RotationSequence=XYX  RotationSequenceAngles=[0 0 0]  RotationSequenceAnglesUnits=deg  RotationMatrix=[1 0 0; 0 1 0; 0 0 1]  Quaternion=[1 0 0 0]  TranslationMethod=StandardAxis  TranslationCartesianOffset=[0 0 0]  TranslationCartesianOffsetUnits=m  TranslationStandardAxis=+X  TranslationStandardOffset=-0.5  TranslationStandardOffsetUnits=m  TranslationROffset=0  TranslationROffsetUnits=m  TranslationThetaOffset=0  TranslationThetaOffsetUnits=deg  TranslationZOffset=0  TranslationZOffsetUnits=m
  Transform Wall Ref pX : sm_lib/Frames and Transforms/Rigid Transform  RotationMethod=StandardAxis  FollAlignAxisA=+X  BaseAlignAxisA=+Y  FollAlignAxisB=+Y  BaseAlignAxisB=+Z  RotationStandardAxis=+Z  RotationAngle=-90  RotationAngleUnits=deg  RotationArbitraryAxis=[0 0 1]  RotationSequenceAxes=FollowerAxes  RotationSequence=XYX  RotationSequenceAngles=[0 0 0]  RotationSequenceAnglesUnits=deg  RotationMatrix=[1 0 0; 0 1 0; 0 0 1]  Quaternion=[1 0 0 0]  TranslationMethod=StandardAxis  TranslationCartesianOffset=[0 0 0]  TranslationCartesianOffsetUnits=m  TranslationStandardAxis=+Y  TranslationStandardOffset=0.5  TranslationStandardOffsetUnits=m  TranslationROffset=0  TranslationROffsetUnits=m  TranslationThetaOffset=0  TranslationThetaOffsetUnits=deg  TranslationZOffset=0  TranslationZOffsetUnits=m
  Transform Wall Ref pZ : sm_lib/Frames and Transforms/Rigid Transform  RotationMethod=StandardAxis  FollAlignAxisA=+X  BaseAlignAxisA=+Y  FollAlignAxisB=+Y  BaseAlignAxisB=+Z  RotationStandardAxis=+Z  RotationAngle=180  RotationAngleUnits=deg  RotationArbitraryAxis=[0 0 1]  RotationSequenceAxes=FollowerAxes  RotationSequence=XYX  RotationSequenceAngles=[0 0 0]  RotationSequenceAnglesUnits=deg  RotationMatrix=[1 0 0; 0 1 0; 0 0 1]  Quaternion=[1 0 0 0]  TranslationMethod=StandardAxis  TranslationCartesianOffset=[0 0 0]  TranslationCartesianOffsetUnits=m  TranslationStandardAxis=+X  TranslationStandardOffset=1  TranslationStandardOffsetUnits=m  TranslationROffset=0  TranslationROffsetUnits=m  TranslationThetaOffset=0  TranslationThetaOffsetUnits=deg  TranslationZOffset=0  TranslationZOffsetUnits=m
  CirF : PMIOPort  Side=Left
  LinB : PMIOPort  Port=2  Side=Right
  wires:
  Circle Line Plus Z/1 -> Terminator3/1
  Circle Line Plus X/1 -> Terminator1/1
  Circle Line Minus X/1 -> Terminator/1
  Circle Line Minus Z/1 -> Terminator2/1
  connections:
  Circle Line Minus X/RConn1 -- Transform Wall Ref mX/RConn1
  Transform Wall Ref pX/RConn1 -- Transform Wall Ref mX/LConn1 -- Circle Line Plus X/RConn1
  LinB/RConn1 -- Transform Wall Ref pX/LConn1 -- Transform Wall Ref mZ/LConn1
  Transform Wall Ref pZ/RConn1 -- Circle Line Plus Z/RConn1
  Transform Wall Ref mZ/RConn1 -- Transform Wall Ref pZ/LConn1 -- Circle Line Minus Z/RConn1
  Circle Line Minus Z/LConn1 -- Circle Line Plus Z/LConn1 -- Circle Line Plus X/LConn1 -- Circle Line Minus X/LConn1 -- CirF/RConn1

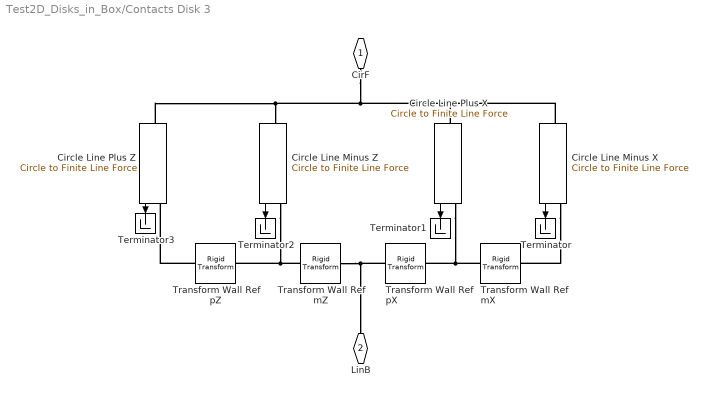
== system Test2D_Disks_in_Box/Contacts Disk 3 ==
  Circle Line Minus X : Contact_Forces_Lib/2D/Circle to Finite Line Force  circle_rad=Disk.radius  line_depth=(Box.outer_width/2-Box.inner_width/2)/2  line_length=(Box.outer_width+Box.inner_width)/2  force_law=Linear  k_contact=k_contact  b_contact=b_contact  pen_full_damp_F=1e-4  pen_exponent=1  custom_param_1=1  custom_param_2=1  friction_law=None  mu_kinetic=0.5  mu_static=0.7  v_thr=0.001  vis_on=off  vis_opc_en=0  vis_len_linBz=Box.width*1.05  vis_len_linBx=Box.outer_width*0.005  vis_len_cirFz=Disk.length*1.05  vis_len_cirFx=Disk.radius*0.05  vis_clr=[0.9 0.2 0.2]  vis_opc=0.7
  Circle Line Minus Z : Contact_Forces_Lib/2D/Circle to Finite Line Force  circle_rad=Disk.radius  line_depth=(Box.outer_width/2-Box.inner_width/2)/2  line_length=(Box.outer_width+Box.inner_width)/2  force_law=Linear  k_contact=k_contact  b_contact=b_contact  pen_full_damp_F=1e-4  pen_exponent=1  custom_param_1=1  custom_param_2=1  friction_law=None  mu_kinetic=0.5  mu_static=0.7  v_thr=0.001  vis_on=off  vis_opc_en=0  vis_len_linBz=Box.width*1.05  vis_len_linBx=Box.outer_width*0.005  vis_len_cirFz=Disk.length*1.05  vis_len_cirFx=Disk.radius*0.05  vis_clr=[0.9 0.2 0.2]  vis_opc=0.7
  Circle Line Plus X : Contact_Forces_Lib/2D/Circle to Finite Line Force  circle_rad=Disk.radius  line_depth=(Box.outer_width/2-Box.inner_width/2)/2  line_length=(Box.outer_width+Box.inner_width)/2  force_law=Linear  k_contact=k_contact  b_contact=b_contact  pen_full_damp_F=1e-4  pen_exponent=1  custom_param_1=1  custom_param_2=1  friction_law=None  mu_kinetic=0.5  mu_static=0.7  v_thr=0.001  vis_on=off  vis_opc_en=0  vis_len_linBz=Box.width*1.05  vis_len_linBx=Box.outer_width*0.005  vis_len_cirFz=Disk.length*1.05  vis_len_cirFx=Disk.radius*0.05  vis_clr=[0.9 0.2 0.2]  vis_opc=0.7
  Circle Line Plus Z : Contact_Forces_Lib/2D/Circle to Finite Line Force  circle_rad=Disk.radius  line_depth=(Box.outer_width/2-Box.inner_width/2)/2  line_length=(Box.outer_width+Box.inner_width)/2  force_law=Linear  k_contact=k_contact  b_contact=b_contact  pen_full_damp_F=1e-4  pen_exponent=1  custom_param_1=1  custom_param_2=1  friction_law=None  mu_kinetic=0.5  mu_static=0.7  v_thr=0.001  vis_on=off  vis_opc_en=0  vis_len_linBz=Box.width*1.05  vis_len_linBx=Box.outer_width*0.005  vis_len_cirFz=Disk.length*1.05  vis_len_cirFx=Disk.radius*0.05  vis_clr=[0.9 0.2 0.2]  vis_opc=0.7
  Terminator{,1..3} (4 alike) : Terminator
  Transform Wall Ref mX : sm_lib/Frames and Transforms/Rigid Transform  RotationMethod=StandardAxis  FollAlignAxisA=+X  BaseAlignAxisA=+Y  FollAlignAxisB=+Y  BaseAlignAxisB=+Z  RotationStandardAxis=+Z  RotationAngle=180  RotationAngleUnits=deg  RotationArbitraryAxis=[0 0 1]  RotationSequenceAxes=FollowerAxes  RotationSequence=XYX  RotationSequenceAngles=[0 0 0]  RotationSequenceAnglesUnits=deg  RotationMatrix=[1 0 0; 0 1 0; 0 0 1]  Quaternion=[1 0 0 0]  TranslationMethod=StandardAxis  TranslationCartesianOffset=[0 0 0]  TranslationCartesianOffsetUnits=m  TranslationStandardAxis=+X  TranslationStandardOffset=1  TranslationStandardOffsetUnits=m  TranslationROffset=0  TranslationROffsetUnits=m  TranslationThetaOffset=0  TranslationThetaOffsetUnits=deg  TranslationZOffset=0  TranslationZOffsetUnits=m
  Transform Wall Ref mZ : sm_lib/Frames and Transforms/Rigid Transform  RotationMethod=None  FollAlignAxisA=+X  BaseAlignAxisA=+Y  FollAlignAxisB=+Y  BaseAlignAxisB=+Z  RotationStandardAxis=+Z  RotationAngle=180  RotationAngleUnits=deg  RotationArbitraryAxis=[0 0 1]  RotationSequenceAxes=FollowerAxes  RotationSequence=XYX  RotationSequenceAngles=[0 0 0]  RotationSequenceAnglesUnits=deg  RotationMatrix=[1 0 0; 0 1 0; 0 0 1]  Quaternion=[1 0 0 0]  TranslationMethod=StandardAxis  TranslationCartesianOffset=[0 0 0]  TranslationCartesianOffsetUnits=m  TranslationStandardAxis=+X  TranslationStandardOffset=-0.5  TranslationStandardOffsetUnits=m  TranslationROffset=0  TranslationROffsetUnits=m  TranslationThetaOffset=0  TranslationThetaOffsetUnits=deg  TranslationZOffset=0  TranslationZOffsetUnits=m
  Transform Wall Ref pX : sm_lib/Frames and Transforms/Rigid Transform  RotationMethod=StandardAxis  FollAlignAxisA=+X  BaseAlignAxisA=+Y  FollAlignAxisB=+Y  BaseAlignAxisB=+Z  RotationStandardAxis=+Z  RotationAngle=-90  RotationAngleUnits=deg  RotationArbitraryAxis=[0 0 1]  RotationSequenceAxes=FollowerAxes  RotationSequence=XYX  RotationSequenceAngles=[0 0 0]  RotationSequenceAnglesUnits=deg  RotationMatrix=[1 0 0; 0 1 0; 0 0 1]  Quaternion=[1 0 0 0]  TranslationMethod=StandardAxis  TranslationCartesianOffset=[0 0 0]  TranslationCartesianOffsetUnits=m  TranslationStandardAxis=+Y  TranslationStandardOffset=0.5  TranslationStandardOffsetUnits=m  TranslationROffset=0  TranslationROffsetUnits=m  TranslationThetaOffset=0  TranslationThetaOffsetUnits=deg  TranslationZOffset=0  TranslationZOffsetUnits=m
  Transform Wall Ref pZ : sm_lib/Frames and Transforms/Rigid Transform  RotationMethod=StandardAxis  FollAlignAxisA=+X  BaseAlignAxisA=+Y  FollAlignAxisB=+Y  BaseAlignAxisB=+Z  RotationStandardAxis=+Z  RotationAngle=180  RotationAngleUnits=deg  RotationArbitraryAxis=[0 0 1]  RotationSequenceAxes=FollowerAxes  RotationSequence=XYX  RotationSequenceAngles=[0 0 0]  RotationSequenceAnglesUnits=deg  RotationMatrix=[1 0 0; 0 1 0; 0 0 1]  Quaternion=[1 0 0 0]  TranslationMethod=StandardAxis  TranslationCartesianOffset=[0 0 0]  TranslationCartesianOffsetUnits=m  TranslationStandardAxis=+X  TranslationStandardOffset=1  TranslationStandardOffsetUnits=m  TranslationROffset=0  TranslationROffsetUnits=m  TranslationThetaOffset=0  TranslationThetaOffsetUnits=deg  TranslationZOffset=0  TranslationZOffsetUnits=m
  CirF : PMIOPort  Side=Left
  LinB : PMIOPort  Port=2  Side=Right
  wires:
  Circle Line Minus Z/1 -> Terminator2/1
  Circle Line Minus X/1 -> Terminator/1
  Circle Line Plus X/1 -> Terminator1/1
  Circle Line Plus Z/1 -> Terminator3/1
  connections:
  CirF/RConn1 -- Circle Line Minus X/LConn1 -- Circle Line Plus X/LConn1 -- Circle Line Plus Z/LConn1 -- Circle Line Minus Z/LConn1
  Circle Line Minus Z/RConn1 -- Transform Wall Ref pZ/LConn1 -- Transform Wall Ref mZ/RConn1
  Transform Wall Ref pZ/RConn1 -- Circle Line Plus Z/RConn1
  Transform Wall Ref mZ/LConn1 -- Transform Wall Ref pX/LConn1 -- LinB/RConn1
  Circle Line Plus X/RConn1 -- Transform Wall Ref mX/LConn1 -- Transform Wall Ref pX/RConn1
  Circle Line Minus X/RConn1 -- Transform Wall Ref mX/RConn1

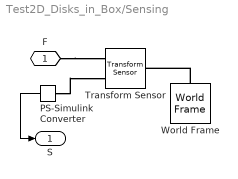
== system Test2D_Disks_in_Box/Sensing ==
  PS-Simulink Converter : nesl_utility/PS-Simulink Converter  PhysicalDomain=network_engine_domain  SubClassName=ps_output  LeftPortType=input  RightPortType=output  PseudoPeriodic=off  Frequencies=[]  VectorFormat=1-D array  Unit=1  AffineConversion=off
  Transform Sensor : sm_lib/Frames and Transforms/Transform Sensor  MeasurementFrame=World  RotationSequence=XYX  SenseAngle=off  SenseAxis=off  SenseQ=off  SenseR=off  SenseRotationSequence=off  SenseOmegaX=off  SenseOmegaY=off  SenseOmegaZ=off  SenseOmega=off  SenseQDot=off  SenseRDot=off  SenseRotationSequenceDot=off  SenseAlphaX=off  SenseAlphaY=off  SenseAlphaZ=off  SenseAlpha=off  SenseQDDot=off  SenseRDDot=off  SenseX=off  SenseY=off  SenseZ=on  SenseXYZ=off  SenseRad=off  SenseAzim=off  SenseDist=off  SenseInc=off  SenseXDot=off  SenseYDot=off  SenseZDot=off  SenseXYZDot=off  SenseRadDot=off  SenseAzimDot=off  SenseDistDot=off  SenseIncDot=off  SenseXDDot=off  SenseYDDot=off  SenseZDDot=off  SenseXYZDDot=off  SenseRadDDot=off  SenseAzimDDot=off  SenseDistDDot=off  SenseIncDDot=off
  World Frame : sm_lib/Frames and Transforms/World Frame
  F : PMIOPort  Side=Left
  S : Outport  VectorParamsAs1DForOutWhenUnconnected=off
  wires:
  PS-Simulink Converter/1 -> S/1
  connections:
  World Frame/RConn1 -- Transform Sensor/LConn1
  F/RConn1 -- Transform Sensor/RConn1
  PS-Simulink Converter/LConn1 -- Transform Sensor/RConn2
